simulink model "ASM_Traffic_MultiCore"  (R2026a)
settings: Solver=ode1  StartTime=SIM.tstart.v  StopTime=SIM.tend.v  FixedStep=SIM.StepSize.v
PostLoadFcn:
  | if any(exist('dsrtsu_mdlpostloadfcn', 'file') ~= 0), dsrtsu_mdlpostloadfcn('Execute', bdroot); end
  | try, asm_mdl_postloadfcn(bdroot, 'UpdateModel', 3600); catch, disp(lasterr); end,
InitFcn:
  | , if any(exist('rtifpga_mdlclblib', 'file') ~= 0), rtifpga_mdlclblib('Init', bdroot); end,
  | , if any(exist('dsmpb_private', 'file') ~= 0), dsmpb_private('dsmpb_mdlclblib', 'Init', bdroot); end,
model workspace (MAT data in the model file):
  asmReferencePath = [0 0.01 0.02 0.03 0.04 0.05 0.06 0.07 0.08 0.09 0.1 0.11 ... (350007 elements, 50001x7)]
  roadBounds : Simulink.Parameter (value not decoded)
  safetyAxes : Simulink.Parameter (value not decoded)
undefined symbols (not defined in the file): _to_, a0b2, ASM_BrakeHydraulics_DemoSystems, ASM_VehicleDynamics_DemoSystems, b98103fe8ad365046cd0, BrakeCircuit, controllerConfig, CPT, Crankshaft, DiscIntNeverNeededParam, dsmsi, FinalDriveAssembly, MDL, ModeSignals, mu, Pos_BrakePedal_Maneuver, rad, RefSignals, roadFamilyData, roadFamilyId, s_to_rpm, SIM, SoftECU, Suspension, Tire, Transmission
libraries: ASM_Traffic_lib x135, simulink x98, ASM_Utils_lib x77, ASM_VehicleDynamics_lib x70, ASM_Environment_lib x22, dsmpblib x20, dsmsilib x15, MDLD_Utils_lib x10, ASM_BrakeHydraulics_lib x3, sl_discontinuities x2
(part 35 of 65)

== system ASM_Traffic_MultiCore/VehicleDynamics/SignalInterface/ExternalOutports/Select_Outport_Signals ==
  ASMSignalBus : Inport
  Bus Selector : BusSelector  OutputSignals=VehicleMovement.Accelerations.VehicleCoG.Linear.a_Vehicle_CoG[x;y;z][m|s2].a_x_Vehicle_CoG[m|s2],VehicleMovement.Accelerations.VehicleCoG.Linear.a_Vehicle_CoG[x;y;z][m|s2].a_y_Vehicle_CoG[m|s2],VehicleMovement.Accelerations.VehicleCoG.Linear.a_Vehicle_CoG[x;y;z][m|s2].a_z_Vehicle_CoG[m|s2],VehicleMovement.Velocities.Vehicle.Linear.v_Vehicle_CoG[x;y;z][km|h].v_x_Vehicle_CoG[km|h],VehicleMovement.Velocities.Vehicle.Linear.v_Vehicle_CoG[x;y;z][km|h].v_y_Vehicle_CoG[km|h],VehicleMovement.Velocities.Vehicle.Linear.v_Vehicle_CoG[x;y;z][km|h].v_z_Vehicle_CoG[km|h],VehicleMovement.Velocities.Vehicle.Linear.v_Total_Vehicle[km|h],VehicleMovement.Velocities.Vehicle.Linear.Angle_SideSlip_Vehicle[deg],VehicleMovement.Velocities.Vehicle.Angular.w_Vehicle_CoG[x;y;z][deg|s].RollRate_Vehicle_CoG[deg|s],VehicleMovement.Velocities.Vehicle.Angular.w_Vehicle_CoG[x;y;z][deg|s].PitchRate_Vehicle_CoG[deg|s],VehicleMovement.Velocities.Vehicle.Angular.w_Vehicle_CoG[x;y;z][deg|s].YawRate_Vehicle_CoG[deg|s],VehicleMovement.Positions.Vehicle.Linear.Pos_Vehicle_CoorSys_E[x;y;z][m].Pos_x_Vehicle_CoorSys_E[m],VehicleMovement.Positions.Vehicle.Linear.Pos_Vehicle_CoorSys_E[x;y;z][m].Pos_y_Vehicle_CoorSys_E[m],VehicleMovement.Positions.Vehicle.Linear.Pos_Vehicle_CoorSys_E[x;y;z][m].Pos_z_Vehicle_CoorSys_E[m],VehicleMovement.Positions.Vehicle.Linear.Pos_Vehicle_CoorSys_E[m],VehicleMovement.Positions.Vehicle.Linear.s_Vehicle[m],VehicleMovement.Positions.Vehicle.Angular.Angle_Vehicle_CoorSys_E[x;y;z][deg].Angle_Roll_Vehicle_CoorSys_E[deg],VehicleMovement.Positions.Vehicle.Angular.Angle_Vehicle_CoorSys_E[x;y;z][deg].Angle_Pitch_Vehicle_CoorSys_E[deg],VehicleMovement.Positions.Vehicle.Angular.Angle_Vehicle_CoorSys_E[x;y;z][deg].Angle_Yaw_Vehicle_CoorSys_E[deg],VehicleMovement.VehicleMassAndAdditionalLoads.m_TotalVehicle[kg],VehicleMovement.VehicleMassAndAdditionalLoads.PosVec_CoG_TotalVehicle[x;y;z][m]  OutputAsBus=on
  Bus Selector1 : BusSelector  OutputSignals=Wheel.WheelSpeed  OutputAsBus=on
  Bus Selector2 : BusSelector  OutputSignals=Brake.BrakeDisc.Pressure,Brake.BrakeDisc.Const_BrakeDiscFactor,Brake.BrakeDisc.Torque  OutputAsBus=on
  Bus Selector3 : BusSelector  OutputSignals=Steering.StatesSteeringSystem,Steering.SteeringWheelTorque,Steering.ForcesAndTorques,Steering.i_Steering_Mean[]  OutputAsBus=on
  Bus Selector4 : BusSelector  OutputSignals=Tire.r_Dyn_Tire[FL;FR;RL;RR][m],Tire.r_Dyn_Tire_Mean[m],Tire.Coef_RollingRes[FL;FR;RL;RR][],Tire.Coef_RollingRes_Mean[],Tire.CorneringStiffness_Tire_Front[N|rad],Tire.CorneringStiffness_Tire_Rear[N|rad],Tire.CorneringStiffness[FL;FR;RL;RR][N|rad]  OutputAsBus=on
  Bus Selector5 : BusSelector  OutputSignals=Suspension.SuspensionFront.RelativePositionFront.Pos_Wheel[FL;FR][x;y;z][m],Suspension.SuspensionRear.RelativePositionRear.Pos_Wheel[RL;RR][x;y;z][m],Suspension.SuspensionFront.SuspensionKinematicsFront,Suspension.SuspensionRear.SuspensionKinematicsRear  OutputAsBus=on
  Bus Selector6 : BusSelector  OutputSignals=Aerodynamics  OutputAsBus=on
  Vehicle_Movement : Outport  VectorParamsAs1DForOutWhenUnconnected=off
  Tire : Outport  Port=2  VectorParamsAs1DForOutWhenUnconnected=off
  WheelSpeed : Outport  Port=3  VectorParamsAs1DForOutWhenUnconnected=off
  Brake : Outport  Port=4  VectorParamsAs1DForOutWhenUnconnected=off
  Steering : Outport  Port=5  VectorParamsAs1DForOutWhenUnconnected=off
  Suspension : Outport  Port=6  VectorParamsAs1DForOutWhenUnconnected=off
  Aerodynamics : Outport  Port=7  VectorParamsAs1DForOutWhenUnconnected=off
  wires:
  Bus Selector3/1 -> Steering/1
  Bus Selector2/1 -> Brake/1
  Bus Selector1/1 -> WheelSpeed/1
  Bus Selector/1 -> Vehicle_Movement/1
  Bus Selector4/1 -> Tire/1
  ASMSignalBus/1 -> Bus Selector/1, Bus Selector4/1, Bus Selector1/1, Bus Selector6/1, Bus Selector5/1, Bus Selector3/1, Bus Selector2/1
  Bus Selector6/1 -> Aerodynamics/1
  Bus Selector5/1 -> Suspension/1

== system ASM_Traffic_MultiCore/AnimationInterface/ANIMATION_INTERFACE/Connection_Settings/Ethernet_TCP/HIL ==
  Tx_Length : Inport
  Tx_Data : Inport  Port=2
  Receive [ETH TCP (Server)\Connection 1] : dsmpblib/Data Inport  Priority=10000
      settings: SourceProductName=dSPACE Model Interface Package for Simulink (MIPS)
  Status [ETH TCP (Server)\Connection 1] : dsmpblib/Data Inport  Priority=10000
      settings: SourceProductName=dSPACE Model Interface Package for Simulink (MIPS)
  Transmit_In [ETH TCP (Server)\Connection 1] : dsmpblib/Data Inport  Priority=10000
      settings: SourceProductName=dSPACE Model Interface Package for Simulink (MIPS)
  Transmit_Out [ETH TCP (Server)\Connection 1] : dsmpblib/Data Outport  Priority=20000
      settings: SourceProductName=dSPACE Model Interface Package for Simulink (MIPS)
  Connected : Outport
  Tx_Sent_bytes : Outport  Port=2
  Rx_Length : Outport  Port=3
  Rx_Data : Outport  Port=4
  wires:
  Tx_Length/1 -> Transmit_Out [ETH TCP (Server)\Connection 1]/1
  Tx_Data/1 -> Transmit_Out [ETH TCP (Server)\Connection 1]/2
  Status [ETH TCP (Server)\Connection 1]/1 -> Connected/1
  Transmit_In [ETH TCP (Server)\Connection 1]/1 -> Tx_Sent_bytes/1
  Receive [ETH TCP (Server)\Connection 1]/1 -> Rx_Length/1
  Receive [ETH TCP (Server)\Connection 1]/2 -> Rx_Data/1

== system ASM_Traffic_MultiCore/AnimationInterface/ANIMATION_INTERFACE/Connection_Settings/Ethernet_TCP/SIL ==
  Tx_Length : Inport
  Tx_Data : Inport  Port=2
  Connected_ : Constant  OutDataTypeStr=Inherit: Inherit via back propagation
  Data Type Conversion : DataTypeConversion  OutDataTypeStr=uint32  SaturateOnIntegerOverflow=off  RndMeth=Floor
  Display : Display
      settings: Format=decimal (Stored Integer)
  dsmsi_eth_tcp_server_BL1 : dsmsilib/Utilities/dsmsi_eth_tcp_server_BL1  paramPort=2017  paramMaximumRxMessageSize=65507  paramBlocking=0  paramEnableReconnectPort=off  paramEnableMaxRxLength=off
      settings: SourceProductName=dSPACE MSI Blockset
  Connected : Outport
  Tx_Sent_bytes : Outport  Port=2
  Rx_Length : Outport  Port=3
  Rx_Data : Outport  Port=4
  wires:
  Data Type Conversion/1 -> Rx_Length/1
  dsmsi_eth_tcp_server_BL1/3 -> Data Type Conversion/1
  Connected_/1 -> Connected/1
  dsmsi_eth_tcp_server_BL1/2 -> Tx_Sent_bytes/1
  dsmsi_eth_tcp_server_BL1/4 -> Rx_Data/1
  dsmsi_eth_tcp_server_BL1/1 -> Display/1
  Tx_Length/1 -> dsmsi_eth_tcp_server_BL1/1
  Tx_Data/1 -> dsmsi_eth_tcp_server_BL1/2

== system ASM_Traffic_MultiCore/AnimationInterface/ANIMATION_INTERFACE/Sensors/Object_Sensor_2D_Points/Calc_Object_Sensor_2D_Points ==
  Transform_In : Inport
  ModelSignals : Inport  Port=2
  Bus Selector2 : BusSelector  OutputSignals=Angle_Hor_Rel[deg],Distance[m],Num_SensorRays_Used[]
  Sensor_Points : Subsystem
  AnimationSignals : Outport  VectorParamsAs1DForOutWhenUnconnected=off
  wires:
  ModelSignals/1 -> Bus Selector2/1
  Transform_In/1 -> Sensor_Points/1(Transform_In)
  Bus Selector2/2 -> Sensor_Points/3(Distance[m])  "<Distance[m]>"
  Sensor_Points/1(Translate[x;y;z][m]) -> AnimationSignals/1
  Bus Selector2/3 -> Sensor_Points/4(Num_SensorRays_Used[])  "<Num_SensorRays_Used[]>"
  Bus Selector2/1 -> Sensor_Points/2(Angle_Hor_Rel[deg])  "<Angle_Hor_Rel[deg]>"

== system ASM_Traffic_MultiCore/AnimationInterface/ANIMATION_INTERFACE/Sensors/Object_Sensor_2D_Points/Object_Sensor_2D_Transformation1 ==
  Transform_In1 : Inport
  ModelSignals : Inport  Port=2
  Bus Selector1 : BusSelector  OutputSignals=Pos_Sensor_Apex_CoorSys_V[x;y;z][m],Angle_z_Orientation_Sensor_CoorSys_V[deg]
  Mux : Mux  Inputs=3
  SensorApex : dsmsilib/dsmsi_simulation_data_objects_BL1  Priority=10001  parameterStr="{\"Version\":1,\"TransformInput\":false,\"EnableInput\":false,\"Objects\":[{\"Name\":\"SensorApex\",\"TypeClass\":{\"Name\":\"Transformation\",\"Class\":1,\"SignalProperty\":null,\"TransformationProperty\":{\"TransformMatrixIn\":true,\"TransformMatrixOut\":true,\"AngleInterpretation\":0,\"TransformationOrder\":0,\"RotationOrder\":0,\"TranslationAsParameter\":false,\"Translation\":\"[0 0 0]\",\"RotationAsParameter\":false,\"Rotation\":\"[0 0 0]\",\"ScalingAsParameter\":true,\"Scaling\":\"[1 1 1]\",\"ObjectsCount\":1},\"PositionAndScaleProperty\":null,\"PositionProperty\":null},\"Children\":[],\"Oid\":1}]}"  evalStr=dsmsi(gcb, 'EvalJson')  sampleTime=-1  globalBlockId=0  objectsBlockId=dsmsi(gcb, 'GetObjectBlockId')  objectsBlockGuiOpen=dsmsi(gcb, 'GetSdoGuiStatus')  dialogIsOpen=0  blockVersion=60  highPrecision=0  validNameBckp=SensorApex
      settings: SourceProductName=dSPACE MSI Blockset
  zero : Constant  Value=0
  Transform_Out : Outport  VectorParamsAs1DForOutWhenUnconnected=off
  wires:
  SensorApex/1 -> Transform_Out/1
  Mux/1 -> SensorApex/3
  Bus Selector1/1 -> SensorApex/2  "<Pos_Sensor_Apex_CoorSys_V[x;y;z][m]>"
  Transform_In1/1 -> SensorApex/1
  ModelSignals/1 -> Bus Selector1/1
  zero/1 -> Mux/3, Mux/2
  Bus Selector1/2 -> Mux/1  "<Angle_z_Orientation_Sensor_CoorSys_V[deg]>"

== system ASM_Traffic_MultiCore/AnimationInterface/ANIMATION_INTERFACE/Sensors/Object_Sensor_3D_CustomPoints/AdaptPointSensor1_To_Dim_60 ==
  ID[] : Inport
  Pos_ObjectPoint_CoorSys_E[x;y;z][m] : Inport  Port=2
  Demux1 : Demux  Outputs=3
  Mux1 : Mux  Inputs=3
  Select_1_60_{1..4} (4 alike) : Selector  InputPortWidth=MDL.Traffic.Sensors.CustomPoints_1.Const_Output_Dimension_Object_Points.v*MDL.Traffic.Sensors.CustomPoints_1.Const_Output_Dimension_Objects.v  IndexOptions=Index vector (dialog)  Indices=[1:60]  OutputSizes=1
  ID_Adatpted[] : Outport  VectorParamsAs1DForOutWhenUnconnected=off
  Pos_ObjectPoint_CoorSys_E_Adapted[x;y;z][m] : Outport  Port=2  VectorParamsAs1DForOutWhenUnconnected=off
  wires:
  Mux1/1 -> Pos_ObjectPoint_CoorSys_E_Adapted[x;y;z][m]/1
  Demux1/3 -> Select_1_60_4/1
  Select_1_60_4/1 -> Mux1/3
  Select_1_60_3/1 -> Mux1/2
  Demux1/2 -> Select_1_60_3/1
  Demux1/1 -> Select_1_60_2/1
  Select_1_60_2/1 -> Mux1/1
  Select_1_60_1/1 -> ID_Adatpted[]/1
  ID[]/1 -> Select_1_60_1/1
  Pos_ObjectPoint_CoorSys_E[x;y;z][m]/1 -> Demux1/1

== system ASM_Traffic_MultiCore/AnimationInterface/ANIMATION_INTERFACE/Sensors/Object_Sensor_3D_CustomPoints/AdaptPointSensor2_To_Dim_60 ==
  ID[] : Inport
  Pos_ObjectPoint_CoorSys_E[x;y;z][m] : Inport  Port=2
  Demux1 : Demux  Outputs=3
  Mux1 : Mux  Inputs=3
  Select_1_60_{1..4} (4 alike) : Selector  InputPortWidth=MDL.Traffic.Sensors.CustomPoints_2.Const_Output_Dimension_Object_Points.v*MDL.Traffic.Sensors.CustomPoints_2.Const_Output_Dimension_Objects.v  IndexOptions=Index vector (dialog)  Indices=[1:60]  OutputSizes=1
  ID_Adatpted[] : Outport  VectorParamsAs1DForOutWhenUnconnected=off
  Pos_ObjectPoint_CoorSys_E_Adapted[x;y;z][m] : Outport  Port=2  VectorParamsAs1DForOutWhenUnconnected=off
  wires:
  Select_1_60_4/1 -> Mux1/3
  Select_1_60_3/1 -> Mux1/2
  Select_1_60_2/1 -> Mux1/1
  Select_1_60_1/1 -> ID_Adatpted[]/1
  Demux1/1 -> Select_1_60_2/1
  Mux1/1 -> Pos_ObjectPoint_CoorSys_E_Adapted[x;y;z][m]/1
  Pos_ObjectPoint_CoorSys_E[x;y;z][m]/1 -> Demux1/1
  ID[]/1 -> Select_1_60_1/1
  Demux1/3 -> Select_1_60_4/1
  Demux1/2 -> Select_1_60_3/1

== system ASM_Traffic_MultiCore/AnimationInterface/ANIMATION_INTERFACE/Sensors/Object_Sensor_3D_CustomPoints/AdaptPointSensor3_To_Dim_60 ==
  ID[] : Inport
  Pos_ObjectPoint_CoorSys_E[x;y;z][m] : Inport  Port=2
  Demux1 : Demux  Outputs=3
  Mux1 : Mux  Inputs=3
  Select_1_60_{1..4} (4 alike) : Selector  InputPortWidth=MDL.Traffic.Sensors.CustomPoints_3.Const_Output_Dimension_Object_Points.v*MDL.Traffic.Sensors.CustomPoints_3.Const_Output_Dimension_Objects.v  IndexOptions=Index vector (dialog)  Indices=[1:60]  OutputSizes=1
  ID_Adatpted[] : Outport  VectorParamsAs1DForOutWhenUnconnected=off
  Pos_ObjectPoint_CoorSys_E_Adapted[x;y;z][m] : Outport  Port=2  VectorParamsAs1DForOutWhenUnconnected=off
  wires:
  Select_1_60_4/1 -> Mux1/3
  Select_1_60_3/1 -> Mux1/2
  Select_1_60_2/1 -> Mux1/1
  Select_1_60_1/1 -> ID_Adatpted[]/1
  Demux1/2 -> Select_1_60_3/1
  Demux1/3 -> Select_1_60_4/1
  ID[]/1 -> Select_1_60_1/1
  Pos_ObjectPoint_CoorSys_E[x;y;z][m]/1 -> Demux1/1
  Mux1/1 -> Pos_ObjectPoint_CoorSys_E_Adapted[x;y;z][m]/1
  Demux1/1 -> Select_1_60_2/1

== system ASM_Traffic_MultiCore/AnimationInterface/ANIMATION_INTERFACE/Sensors/Object_Sensor_3D_RadarEffect_Points/AdaptPointDimensionSensor1 ==
  ID[] : Inport
  Pos_ObjectPoint_CoorSys_E[x;y;z][m] : Inport  Port=2
  Demux1 : Demux  Outputs=3
  Mux1 : Mux  Inputs=3
  Selector{1..4} (4 alike) : Selector  InputPortWidth=MDL.Traffic.Sensors.RadarReflectionPoints_1.Const_Output_Dimension_Objects.v*MDL.Traffic.Sensors.RadarReflectionPoints_1.Const_Output_Dimension_Object_Points.v  IndexOptions=Index vector (dialog)  Indices=[1:60]  OutputSizes=1
  ID_Adatpted[] : Outport  VectorParamsAs1DForOutWhenUnconnected=off
  Pos_ObjectPoint_CoorSys_E_Adapted[x;y;z][m] : Outport  Port=2  VectorParamsAs1DForOutWhenUnconnected=off
  wires:
  Pos_ObjectPoint_CoorSys_E[x;y;z][m]/1 -> Demux1/1
  ID[]/1 -> Selector3/1
  Selector3/1 -> ID_Adatpted[]/1
  Selector1/1 -> Mux1/1
  Demux1/1 -> Selector1/1
  Demux1/2 -> Selector2/1
  Selector2/1 -> Mux1/2
  Selector4/1 -> Mux1/3
  Demux1/3 -> Selector4/1
  Mux1/1 -> Pos_ObjectPoint_CoorSys_E_Adapted[x;y;z][m]/1

== system ASM_Traffic_MultiCore/AnimationInterface/ANIMATION_INTERFACE/Sensors/Object_Sensor_3D_RadarEffect_Points/AdaptPointDimensionSensor2 ==
  ID[] : Inport
  Pos_ObjectPoint_CoorSys_E[x;y;z][m] : Inport  Port=2
  Demux1 : Demux  Outputs=3
  Mux1 : Mux  Inputs=3
  Selector{1..4} (4 alike) : Selector  InputPortWidth=MDL.Traffic.Sensors.RadarReflectionPoints_2.Const_Output_Dimension_Objects.v*MDL.Traffic.Sensors.RadarReflectionPoints_2.Const_Output_Dimension_Object_Points.v  IndexOptions=Index vector (dialog)  Indices=[1:60]  OutputSizes=1
  ID_Adatpted[] : Outport  VectorParamsAs1DForOutWhenUnconnected=off
  Pos_ObjectPoint_CoorSys_E_Adapted[x;y;z][m] : Outport  Port=2  VectorParamsAs1DForOutWhenUnconnected=off
  wires:
  Mux1/1 -> Pos_ObjectPoint_CoorSys_E_Adapted[x;y;z][m]/1
  Demux1/3 -> Selector4/1
  Selector4/1 -> Mux1/3
  Selector2/1 -> Mux1/2
  Demux1/2 -> Selector2/1
  Demux1/1 -> Selector1/1
  Selector1/1 -> Mux1/1
  Selector3/1 -> ID_Adatpted[]/1
  ID[]/1 -> Selector3/1
  Pos_ObjectPoint_CoorSys_E[x;y;z][m]/1 -> Demux1/1

== system ASM_Traffic_MultiCore/AnimationInterface/ANIMATION_INTERFACE/Sensors/Object_Sensor_3D_RadarEffect_Points/AdaptPointDimensionSensor3 ==
  ID[] : Inport
  Pos_ObjectPoint_CoorSys_E[x;y;z][m] : Inport  Port=2
  Demux1 : Demux  Outputs=3
  Mux1 : Mux  Inputs=3
  Selector{1..4} (4 alike) : Selector  InputPortWidth=MDL.Traffic.Sensors.RadarReflectionPoints_3.Const_Output_Dimension_Objects.v*MDL.Traffic.Sensors.RadarReflectionPoints_3.Const_Output_Dimension_Object_Points.v  IndexOptions=Index vector (dialog)  Indices=[1:60]  OutputSizes=1
  ID_Adatpted[] : Outport  VectorParamsAs1DForOutWhenUnconnected=off
  Pos_ObjectPoint_CoorSys_E_Adapted[x;y;z][m] : Outport  Port=2  VectorParamsAs1DForOutWhenUnconnected=off
  wires:
  Pos_ObjectPoint_CoorSys_E[x;y;z][m]/1 -> Demux1/1
  ID[]/1 -> Selector3/1
  Selector3/1 -> ID_Adatpted[]/1
  Selector1/1 -> Mux1/1
  Demux1/1 -> Selector1/1
  Demux1/2 -> Selector2/1
  Selector2/1 -> Mux1/2
  Selector4/1 -> Mux1/3
  Demux1/3 -> Selector4/1
  Mux1/1 -> Pos_ObjectPoint_CoorSys_E_Adapted[x;y;z][m]/1

== system ASM_Traffic_MultiCore/DomainControl/DriverAssistance/Control/SoftECU_ACC/Soft_ECU_ACC ==
  Switches_ACC_User : Inport
  v_x_Vehicle_CoG[km|h] : Inport  Port=2
  YawRate_Vehicle_CoG[deg|s] : Inport  Port=3
  Pos_FL_Wheel[x;y;z][m] : Inport  Port=4
  Pos_FR_Wheel[x;y;z][m] : Inport  Port=5
  r_Dyn_Tire[FL;FR;RL;RR][m] : Inport  Port=6
  Coef_RollingRes[FL;FR;RL;RR][] : Inport  Port=7
  Cw_x[] : Inport  Port=8
  i_FrontDrive[] : Inport  Port=9
  i_RearDrive[] : Inport  Port=10
  TrqDistri_Front_Rear[0_1] : Inport  Port=11
  i_unsync_Trm[] : Inport  Port=12
  m_TotalVehicle[kg] : Inport  Port=13
  Trq_Fric_Engine[Nm] : Inport  Port=14
  Pos_AccPedal[%] : Inport  Port=15
  Pos_BrakePedal[%] : Inport  Port=16
  Slope_Veh_Road[%] : Inport  Port=17
  s_Vehicle_Road[m] : Inport  Port=18
  d_Vehicle_Road[m] : Inport  Port=19
  Dist_Fellows[m] : Inport  Port=20
  v_Rel_Fellows[m|s] : Inport  Port=21
  Angle_Hor_Rel_Fellows[deg] : Inport  Port=22
  s_Fellows_Ref[m] : Inport  Port=23
  d_Total_Fellows[m] : Inport  Port=24
  PosVec_MainPnt_Fellows[x;y;z][m] : Inport  Port=25
  Length_Fellows[m] : Inport  Port=26
  Width_Fellows[m] : Inport  Port=27
  Height_Fellows[m] : Inport  Port=28
  Object_ID[] : Inport  Port=29
  ECU_Commands[] : Inport  Port=30
  Reset[0|1] : Inport  Port=31
  ASMSignalCollector : Subsystem
  CONTROLLER_ACC : ASM_Traffic_lib/SoftECU/CONTROLLER_ACC  Tag=ASM_SUBCOMPONENT  Const_Kp_Dist_Ctrl=MDL.SoftECU.ACC.Const_Kp_Dist_Ctrl  Const_Ki_Dist_Ctrl=MDL.SoftECU.ACC.Const_Ki_Dist_Ctrl  Const_Kp_v_Ctrl=MDL.SoftECU.ACC.Const_Kp_v_Ctrl  Const_Ki_v_Ctrl=MDL.SoftECU.ACC.Const_Ki_v_Ctrl  Map_a_UpperLimit=MDL.SoftECU.ACC.Map_a_UpperLimit  Map_a_LowerLimit=MDL.SoftECU.ACC.Map_a_LowerLimit  Const_v_Threshold=MDL.SoftECU.ACC.Const_v_Threshold  Const_Dist_Threshold=MDL.SoftECU.ACC.Const_Dist_Threshold  Map_a_RisingRateMax=MDL.SoftECU.ACC.Map_a_RisingRateMax  Map_a_FallingRateMax=MDL.SoftECU.ACC.Map_a_FallingRateMax  Const_a_Max_AEB=MDL.SoftECU.ACC.Const_a_Max_AEB  Const_Response_Time_FCW=MDL.SoftECU.ACC.Const_Response_Time_FCW  Const_Dist_Min_Set=MDL.SoftECU.ACC.Const_Dist_Min_Set  Map_TTCThresholdAEB=MDL.SoftECU.ACC.Map_TTCThresholdAEB  StepSize=SIM.StepSize  ASMProperties=struct('Name','CONTROLLER_ACC','Version','9.0','Library','ASM_Traffic_lib')  ASMInstanceName=controller_acc  ASMInstanceID=1
  ControlModel_Signals : Subsystem
  Goto Tag Visibility : GotoTagVisibility  GotoTag=ASMBUS_SoftECU_ACC_Target_Selection
  Goto Tag Visibility1 : GotoTagVisibility  GotoTag=ASMBUS_SoftECU_ACC_Controller
  Goto Tag Visibility2 : GotoTagVisibility  GotoTag=ASMBUS_SoftECU_ACC_User_Interface
  Goto Tag Visibility3 : GotoTagVisibility  GotoTag=ASMBUS_SoftECU_ACC_Interface
  Input_Selection : Subsystem
  Map_Inputs : Subsystem
  Mux : Mux  Inputs=2
  OUTPUT_INTERFACE_ACC : ASM_Traffic_lib/SoftECU/OUTPUT_INTERFACE_ACC  Tag=ASM_SUBCOMPONENT  ASMProperties=struct('Name','OUTPUT_INTERFACE_ACC','Version','5.0','Library','ASM_Traffic_lib')  ASMInstanceName=output_interface_acc  ASMInstanceID=1
  Rate Transition : RateTransition  Integrity=off  OutPortSampleTimeOpt=Inherit
  Rate Transition1 : RateTransition  Integrity=off  OutPortSampleTimeOpt=Inherit
  Sw_ACC_Distance[s] : Constant  Value=2
  TARGET_SELECTION_ACC : ASM_Traffic_lib/SoftECU/TARGET_SELECTION_ACC  Tag=ASM_SUBCOMPONENT  Const_Dist_SafetyBound=MDL.SoftECU.ACC.Const_Dist_SafetyBound  Sw_LaneCrossingCheck=MDL.SoftECU.ACC.Sw_LaneCrossingCheck  StepSize=SIM.StepSize  ASMProperties=struct('Name','TARGET_SELECTION_ACC','Version','6.0','Library','ASM_Traffic_lib')  ASMInstanceName=target_selection_acc  ASMInstanceID=1
  Tire : Subsystem
  TrackWidthVehicle : Subsystem
  USER_INTERFACE_ACC : ASM_Traffic_lib/SoftECU/USER_INTERFACE_ACC  Tag=ASM_SUBCOMPONENT  Const_v_Step=MDL.SoftECU.ACC.Const_v_Step_CC  ASMProperties=struct('Name','USER_INTERFACE_ACC','Version','6.0','Library','ASM_Traffic_lib')  ASMInstanceName=user_interface_acc  ASMInstanceID=1
  avoid_incomplete_trace2source : Subsystem
  avoid_incomplete_trace2source1 : Subsystem
  avoid_incomplete_trace2source10 : Subsystem
  avoid_incomplete_trace2source2 : Subsystem
  avoid_incomplete_trace2source4 : Subsystem
  avoid_incomplete_trace2source5 : Subsystem
  avoid_incomplete_trace2source6 : Subsystem
  avoid_incomplete_trace2source7 : Subsystem
  avoid_incomplete_trace2source8 : Subsystem
  avoid_incomplete_trace2source9 : Subsystem
  hide_algebraic_loop : UnitDelay  SampleTime=-1
  hide_algebraic_loop1 : UnitDelay  SampleTime=-1
  "hide_algebraic_loop2 " : UnitDelay  SampleTime=-1
  ASMSignalBus : Outport  VectorParamsAs1DForOutWhenUnconnected=off
  Enable_Trq_Engine_ACC[0|1] : Outport  Port=2  VectorParamsAs1DForOutWhenUnconnected=off
  Trq_Request_Engine_ACC[Nm] : Outport  Port=3  VectorParamsAs1DForOutWhenUnconnected=off
  Trq_Request_Engine_ACC[Front;Rear][Nm] : Outport  Port=4  VectorParamsAs1DForOutWhenUnconnected=off
  Enable_Trq_Brake_ACC[0|1] : Outport  Port=5  VectorParamsAs1DForOutWhenUnconnected=off
  Trq_Request_Brake_ACC[Nm] : Outport  Port=6  VectorParamsAs1DForOutWhenUnconnected=off
  FCW[0|1] : Outport  Port=7  VectorParamsAs1DForOutWhenUnconnected=off
  AEB[0|1] : Outport  Port=8  VectorParamsAs1DForOutWhenUnconnected=off
  ACC_State[1OFF|2Standby|3ON] : Outport  Port=9  VectorParamsAs1DForOutWhenUnconnected=off
  Driver_Override_ACC_Active[0Off|1On] : Outport  Port=10  VectorParamsAs1DForOutWhenUnconnected=off
  Driver_Override_ACC_Reason[0NoOverride|1BrakePedal|2AccPedal] : Outport  Port=11  VectorParamsAs1DForOutWhenUnconnected=off
  tag scope: ASMBUS_SoftECU_ACC_Controller=scoped, ASMBUS_SoftECU_ACC_Interface=scoped, ASMBUS_SoftECU_ACC_Target_Selection=scoped, ASMBUS_SoftECU_ACC_User_Interface=scoped
  wires:
  avoid_incomplete_trace2source10/1(Out1) -> USER_INTERFACE_ACC/10
  Map_Inputs/7(Sw_ACC_Speed_Decrease[0Off|1On]) -> avoid_incomplete_trace2source10/1(In1)
  avoid_incomplete_trace2source9/1(Out1) -> USER_INTERFACE_ACC/9
  Map_Inputs/6(Sw_ACC_Speed_Increase[0Off|1On]) -> avoid_incomplete_trace2source9/1(In1)
  avoid_incomplete_trace2source8/1(Out1) -> USER_INTERFACE_ACC/8
  Map_Inputs/5(Sw_ACC_Speed_Set[0Off|1On]) -> avoid_incomplete_trace2source8/1(In1)
  avoid_incomplete_trace2source7/1(Out1) -> USER_INTERFACE_ACC/7
  Map_Inputs/4(Sw_ACC_Resume[0Off|1On]) -> avoid_incomplete_trace2source7/1(In1)
  avoid_incomplete_trace2source6/1(Out1) -> USER_INTERFACE_ACC/6
  Map_Inputs/3(Sw_ACC_Cancel[0Off|1On]) -> avoid_incomplete_trace2source6/1(In1)
  avoid_incomplete_trace2source5/1(Out1) -> USER_INTERFACE_ACC/5
  Map_Inputs/2(Sw_ACC_Off[0Off|1On]) -> avoid_incomplete_trace2source5/1(In1)
  avoid_incomplete_trace2source4/1(Out1) -> USER_INTERFACE_ACC/4
  Map_Inputs/1(Sw_ACC_On[0Off|1On]) -> avoid_incomplete_trace2source4/1(In1)
  Sw_ACC_Distance[s]/1 -> CONTROLLER_ACC/10
  avoid_incomplete_trace2source2/1(Out1) -> CONTROLLER_ACC/9
  Map_Inputs/8(Sw_ACC_BrakeMode[1Comfort|2AEBOnly|3AEBOff]) -> avoid_incomplete_trace2source2/1(In1)
  avoid_incomplete_trace2source1/1(Out1) -> CONTROLLER_ACC/8
  USER_INTERFACE_ACC/3 -> avoid_incomplete_trace2source1/1(In1)
  avoid_incomplete_trace2source/1(Out1) -> CONTROLLER_ACC/7
  USER_INTERFACE_ACC/2 -> avoid_incomplete_trace2source/1(In1)
  CONTROLLER_ACC/6 -> AEB[0|1]/1
  CONTROLLER_ACC/5 -> FCW[0|1]/1
  Trq_Fric_Engine[Nm]/1 -> OUTPUT_INTERFACE_ACC/10
  Coef_RollingRes[FL;FR;RL;RR][]/1 -> Tire/2(Coef_RollingRes[FL;FR;RL;RR][])
  r_Dyn_Tire[FL;FR;RL;RR][m]/1 -> Tire/1(r_Dyn_Tire[FL;FR;RL;RR][m])
  CONTROLLER_ACC/1 -> [ASMBUS_SoftECU_ACC_Controller]
  ASMSignalCollector/1(ASMSignalBus) -> ASMSignalBus/1
  Tire/1(r_Dyn_Tire_Mean[m]) -> OUTPUT_INTERFACE_ACC/2
  Tire/2(Coef_RollingRes_Mean[]) -> OUTPUT_INTERFACE_ACC/3
  Cw_x[]/1 -> OUTPUT_INTERFACE_ACC/4
  Slope_Veh_Road[%]/1 -> OUTPUT_INTERFACE_ACC/8
  v_x_Vehicle_CoG[km|h]/1 -> TARGET_SELECTION_ACC/2, USER_INTERFACE_ACC/1, CONTROLLER_ACC/1, OUTPUT_INTERFACE_ACC/9
  OUTPUT_INTERFACE_ACC/3 -> Trq_Request_Engine_ACC[Nm]/1
  OUTPUT_INTERFACE_ACC/2 -> Trq_Request_Brake_ACC[Nm]/1
  OUTPUT_INTERFACE_ACC/1 -> [ASMBUS_SoftECU_ACC_Interface]
  i_unsync_Trm[]/1 -> OUTPUT_INTERFACE_ACC/6
  m_TotalVehicle[kg]/1 -> OUTPUT_INTERFACE_ACC/7
  YawRate_Vehicle_CoG[deg|s]/1 -> TARGET_SELECTION_ACC/1
  CONTROLLER_ACC/2 -> hide_algebraic_loop/1
  TARGET_SELECTION_ACC/1 -> [ASMBUS_SoftECU_ACC_Target_Selection]
  Mux/1 -> OUTPUT_INTERFACE_ACC/5
  USER_INTERFACE_ACC/1 -> [ASMBUS_SoftECU_ACC_User_Interface]
  Switches_ACC_User/1 -> Map_Inputs/2(Switches_ACC_User)
  ECU_Commands[]/1 -> Map_Inputs/3(ECU_Commands[])
  TARGET_SELECTION_ACC/4 -> CONTROLLER_ACC/4
  TARGET_SELECTION_ACC/3 -> CONTROLLER_ACC/3
  TARGET_SELECTION_ACC/2 -> Rate Transition/1
  Rate Transition/1 -> CONTROLLER_ACC/2
  CONTROLLER_ACC/3 -> hide_algebraic_loop1/1
  CONTROLLER_ACC/4 -> "hide_algebraic_loop2 "/1
  hide_algebraic_loop1/1 -> Enable_Trq_Engine_ACC[0|1]/1, OUTPUT_INTERFACE_ACC/11
  "hide_algebraic_loop2 "/1 -> Enable_Trq_Brake_ACC[0|1]/1, OUTPUT_INTERFACE_ACC/12
  hide_algebraic_loop/1 -> OUTPUT_INTERFACE_ACC/1
  Pos_AccPedal[%]/1 -> USER_INTERFACE_ACC/2
  Pos_BrakePedal[%]/1 -> USER_INTERFACE_ACC/3
  Pos_FL_Wheel[x;y;z][m]/1 -> TrackWidthVehicle/1(Pos_FL_Wheel[x;y;z][m])
  Pos_FR_Wheel[x;y;z][m]/1 -> TrackWidthVehicle/2(Pos_FR_Wheel[x;y;z][m])
  TrackWidthVehicle/1(TrackWidth_Vehicle[m]) -> TARGET_SELECTION_ACC/3
  Dist_Fellows[m]/1 -> TARGET_SELECTION_ACC/4
  v_Rel_Fellows[m|s]/1 -> TARGET_SELECTION_ACC/5
  Angle_Hor_Rel_Fellows[deg]/1 -> TARGET_SELECTION_ACC/6
  Reset[0|1]/1 -> Map_Inputs/1(Reset[0|1]), USER_INTERFACE_ACC/11, TARGET_SELECTION_ACC/7
  d_Total_Fellows[m]/1 -> TARGET_SELECTION_ACC/9
  s_Fellows_Ref[m]/1 -> Rate Transition1/1
  s_Vehicle_Road[m]/1 -> TARGET_SELECTION_ACC/10
  d_Vehicle_Road[m]/1 -> TARGET_SELECTION_ACC/11
  Object_ID[]/1 -> TARGET_SELECTION_ACC/16
  TARGET_SELECTION_ACC/5 -> CONTROLLER_ACC/5
  TARGET_SELECTION_ACC/6 -> CONTROLLER_ACC/6
  Length_Fellows[m]/1 -> TARGET_SELECTION_ACC/13
  Width_Fellows[m]/1 -> TARGET_SELECTION_ACC/14
  Height_Fellows[m]/1 -> TARGET_SELECTION_ACC/15
  PosVec_MainPnt_Fellows[x;y;z][m]/1 -> Input_Selection/1(PosVec_MainPnt_Fellows[x;y;z][m])
  Input_Selection/1(Pos_x_MainPnt_Fellows[m]) -> TARGET_SELECTION_ACC/12
  Rate Transition1/1 -> TARGET_SELECTION_ACC/8
  OUTPUT_INTERFACE_ACC/4 -> Trq_Request_Engine_ACC[Front;Rear][Nm]/1
  TrqDistri_Front_Rear[0_1]/1 -> OUTPUT_INTERFACE_ACC/13
  i_FrontDrive[]/1 -> Mux/1
  i_RearDrive[]/1 -> Mux/2
  ControlModel_Signals/1(ACC_State[1OFF|2Standby|3ON]) -> ACC_State[1OFF|2Standby|3ON]/1
  ControlModel_Signals/2(Driver_Override_ACC_Active[0Off|1On]) -> Driver_Override_ACC_Active[0Off|1On]/1
  ControlModel_Signals/3(Driver_Override_ACC_Reason[0NoOverride|1BrakePedal|2AccPedal]) -> Driver_Override_ACC_Reason[0NoOverride|1BrakePedal|2AccPedal]/1

== system ASM_Traffic_MultiCore/DomainControl/DriverAssistance/Control/Sw_ECU_Signals/ACC_State[1OFF|2Standby|3ON] ==
  SoftECU : Inport
  RealECU : Inport  Port=2
  Const_ACC_State[1OFF|2Standby|3ON] : Constant
  MultiPortSwitch : MultiPortSwitch
  Sw_ACC_State[1SoftECU|2RealECU|3Const] : Constant  Value=CPT.MDL_SW.Sw_ACC_State.v
  ACC_State[1OFF|2Standby|3ON] : Outport  VectorParamsAs1DForOutWhenUnconnected=off
  wires:
  MultiPortSwitch/1 -> ACC_State[1OFF|2Standby|3ON]/1
  Const_ACC_State[1OFF|2Standby|3ON]/1 -> MultiPortSwitch/4
  RealECU/1 -> MultiPortSwitch/3
  SoftECU/1 -> MultiPortSwitch/2
  Sw_ACC_State[1SoftECU|2RealECU|3Const]/1 -> MultiPortSwitch/1

== system ASM_Traffic_MultiCore/DomainControl/DriverAssistance/Control/Sw_ECU_Signals/AEB[0|1] ==
  SoftECU : Inport
  RealECU : Inport  Port=2
  Const_AEB[0|1] : Constant  Value=0
  MultiPortSwitch : MultiPortSwitch
  Sw_AEB[1SoftECU|2RealECU|3Const] : Constant  Value=CPT.MDL_SW.Sw_AEB.v
  AEB[0|1] : Outport  VectorParamsAs1DForOutWhenUnconnected=off
  wires:
  MultiPortSwitch/1 -> AEB[0|1]/1
  Const_AEB[0|1]/1 -> MultiPortSwitch/4
  RealECU/1 -> MultiPortSwitch/3
  SoftECU/1 -> MultiPortSwitch/2
  Sw_AEB[1SoftECU|2RealECU|3Const]/1 -> MultiPortSwitch/1

== system ASM_Traffic_MultiCore/DomainControl/DriverAssistance/Control/Sw_ECU_Signals/Enable_Trq_Decrease_ACC[0|1] ==
  SoftECU : Inport
  RealECU : Inport  Port=2
  Const_Enable_Trq_Decrease_ACC[0|1] : Constant  Value=0
  MultiPortSwitch : MultiPortSwitch
  Sw_Enable_Trq_Decrease_ACC[1SoftECU|2RealECU|3Const] : Constant  Value=CPT.MDL_SW.Sw_Enable_Trq_Decrease_ACC.v
  Enable_Trq_Decrease_ACC[0|1] : Outport  VectorParamsAs1DForOutWhenUnconnected=off
  wires:
  MultiPortSwitch/1 -> Enable_Trq_Decrease_ACC[0|1]/1
  Const_Enable_Trq_Decrease_ACC[0|1]/1 -> MultiPortSwitch/4
  RealECU/1 -> MultiPortSwitch/3
  SoftECU/1 -> MultiPortSwitch/2
  Sw_Enable_Trq_Decrease_ACC[1SoftECU|2RealECU|3Const]/1 -> MultiPortSwitch/1

== system ASM_Traffic_MultiCore/DomainControl/DriverAssistance/Control/Sw_ECU_Signals/Enable_Trq_Increase_ACC[0|1] ==
  SoftECU : Inport
  RealECU : Inport  Port=2
  Const_Enable_Trq_Increase_ACC[0|1] : Constant  Value=0
  MultiPortSwitch : MultiPortSwitch
  Sw_Enable_Trq_Increase_ACC[1SoftECU|2RealECU|3Const] : Constant  Value=CPT.MDL_SW.Sw_Enable_Trq_Increase_ACC.v
  Enable_Trq_Increase_ACC[0|1] : Outport  VectorParamsAs1DForOutWhenUnconnected=off
  wires:
  Sw_Enable_Trq_Increase_ACC[1SoftECU|2RealECU|3Const]/1 -> MultiPortSwitch/1
  SoftECU/1 -> MultiPortSwitch/2
  RealECU/1 -> MultiPortSwitch/3
  Const_Enable_Trq_Increase_ACC[0|1]/1 -> MultiPortSwitch/4
  MultiPortSwitch/1 -> Enable_Trq_Increase_ACC[0|1]/1

== system ASM_Traffic_MultiCore/DomainControl/DriverAssistance/Control/Sw_ECU_Signals/FCW[0|1] ==
  SoftECU : Inport
  RealECU : Inport  Port=2
  Const_FCW[0|1] : Constant  Value=0
  MultiPortSwitch : MultiPortSwitch
  Sw_FCW[1SoftECU|2RealECU|3Const] : Constant  Value=CPT.MDL_SW.Sw_FCW.v
  FCW[0|1] : Outport  VectorParamsAs1DForOutWhenUnconnected=off
  wires:
  MultiPortSwitch/1 -> FCW[0|1]/1
  Const_FCW[0|1]/1 -> MultiPortSwitch/4
  RealECU/1 -> MultiPortSwitch/3
  SoftECU/1 -> MultiPortSwitch/2
  Sw_FCW[1SoftECU|2RealECU|3Const]/1 -> MultiPortSwitch/1

== system ASM_Traffic_MultiCore/DomainControl/DriverAssistance/Control/Sw_ECU_Signals/Trq_DecreaseRequest_ACC[Nm] ==
  SoftECU : Inport
  RealECU : Inport  Port=2
  Const_Trq_DecreaseRequest_ACC[Nm] : Constant  Value=0
  MultiPortSwitch : MultiPortSwitch
  Sw_Trq_DecreaseRequest_ACC[1SoftECU|2RealECU|3Const] : Constant  Value=CPT.MDL_SW.Sw_Trq_DecreaseRequest_ACC.v
  Trq_DecreaseRequest_ACC[Nm] : Outport  VectorParamsAs1DForOutWhenUnconnected=off
  wires:
  MultiPortSwitch/1 -> Trq_DecreaseRequest_ACC[Nm]/1
  Const_Trq_DecreaseRequest_ACC[Nm]/1 -> MultiPortSwitch/4
  RealECU/1 -> MultiPortSwitch/3
  SoftECU/1 -> MultiPortSwitch/2
  Sw_Trq_DecreaseRequest_ACC[1SoftECU|2RealECU|3Const]/1 -> MultiPortSwitch/1

== system ASM_Traffic_MultiCore/DomainControl/DriverAssistance/Control/Sw_ECU_Signals/Trq_IncreaseRequest_ACC[Front;Rear][Nm] ==
  SoftECU : Inport
  RealECU : Inport  Port=2
  Const_Trq_IncreaseRequest_ACC[Front;Rear][Nm] : Constant  Value=[0;0]
  MultiPortSwitch : MultiPortSwitch
  Sw_Trq_IncreaseRequest_ACC[Front;Rear][1SoftECU|2RealECU|3Const] : Constant  Value=CPT.MDL_SW.Sw_Trq_IncreaseRequest_ACC.v
  Trq_IncreaseRequest_ACC[Front;Rear][Nm] : Outport  VectorParamsAs1DForOutWhenUnconnected=off
  wires:
  Sw_Trq_IncreaseRequest_ACC[Front;Rear][1SoftECU|2RealECU|3Const]/1 -> MultiPortSwitch/1
  SoftECU/1 -> MultiPortSwitch/2
  RealECU/1 -> MultiPortSwitch/3
  Const_Trq_IncreaseRequest_ACC[Front;Rear][Nm]/1 -> MultiPortSwitch/4
  MultiPortSwitch/1 -> Trq_IncreaseRequest_ACC[Front;Rear][Nm]/1

== system ASM_Traffic_MultiCore/DomainControl/DriverAssistance/Control/Sw_ECU_Signals/Trq_IncreaseRequest_ACC[Nm] ==
  SoftECU : Inport
  RealECU : Inport  Port=2
  Const_Trq_IncreaseRequest_ACC[Nm] : Constant  Value=0
  MultiPortSwitch : MultiPortSwitch
  Sw_Trq_IncreaseRequest_ACC[1SoftECU|2RealECU|3Const] : Constant  Value=CPT.MDL_SW.Sw_Trq_IncreaseRequest_ACC.v
  Trq_IncreaseRequest_ACC[Nm] : Outport  VectorParamsAs1DForOutWhenUnconnected=off
  wires:
  Sw_Trq_IncreaseRequest_ACC[1SoftECU|2RealECU|3Const]/1 -> MultiPortSwitch/1
  SoftECU/1 -> MultiPortSwitch/2
  RealECU/1 -> MultiPortSwitch/3
  Const_Trq_IncreaseRequest_ACC[Nm]/1 -> MultiPortSwitch/4
  MultiPortSwitch/1 -> Trq_IncreaseRequest_ACC[Nm]/1

== system ASM_Traffic_MultiCore/DomainControl/DriverAssistance/Control/UserInterface/ASMSignalBus_Control ==
  In : Inport
  Terminator_1 : Terminator
  tag scope: ASMBUS_DriverAssistance_Control=global
  wires:
  [ASMBUS_DriverAssistance_Control] -> Terminator_1/1
  In/1 -> [ASMBUS_DriverAssistance_Control]  "Control"

== system ASM_Traffic_MultiCore/DomainControl/DriverAssistance/Control/UserInterface/DISP_Control ==
  Interface_In : Inport
  In : Inport  Port=2
  ACC_Control_Mode[0OFF|1CC|2DC] : Subsystem
      mask Display: disp('')
  ACC_State[0OFF|2Standby|3ON] : Subsystem
      mask Display: disp('')
  AEB[0Off|1On] : Subsystem
      mask Display: disp('')
  Bus Selector1 : BusSelector  OutputSignals=Controller_ACC.State_ACC[0Off|1On],Controller_ACC.Control_Mode_ACC[0Off|1CC|2DC],Controller_ACC.FCW[0Off|1On],Controller_ACC.AEB[0Off|1On],Controller_ACC.TTC[s],Controller_ACC.Collision[0Off|1On],Controller_ACC.Sw_BrakeMode[1Comfort|2AEBOnly|3AEBOff]
  Bus Selector3 : BusSelector  OutputSignals=Controller_ACC.Control_Mode_ACC[0Off|1CC|2DC],Controller_ACC.v_Set[km|h],Target_Selection_ACC.v_Rel[m|s],Controller_ACC.Distance_Set[m],Target_Selection_ACC.Dist_Long[m],Interface_ACC.Trq_Request_Brake_ACC[Nm],Interface_ACC.Trq_Request_Engine_ACC[Nm],Operator_Interface_ACC.ACC_State[1OFF|2Standby|3ON],Target_Selection_ACC.Target_Detected[0|1]
  Bus Selector5 : BusSelector  OutputSignals=ExternalModel.v_Vehicle[km|h]
  Collision[0Off|1On] : Subsystem
      mask Display: disp('')
  Control_Mode_ACC[0Off|1CC|2DC] : Subsystem
      mask Display: disp('')
  Dist_Long[m] : Subsystem
      mask Display: disp('')
  Distance_Set[m] : Subsystem
      mask Display: disp('')
  FCW[0Off|1On] : Subsystem
      mask Display: disp('')
  Mux1 : Mux  Inputs=2
  Mux3 : Mux  Inputs=2
  SoftECU_ACC_Info : Scope  NumInputPorts=6
      settings: TimeSpan=5  ActiveDisplayYMinimum=-0.25  ActiveDisplayYMaximum=2.25  DataLoggingMaxPoints=20000  DataLoggingDecimation=10
  SoftECU_ACC_States : Scope  NumInputPorts=7
      settings: TimeSpan=5  ActiveDisplayYMinimum=-0.125  ActiveDisplayYMaximum=1.125  DataLoggingMaxPoints=20000  DataLoggingDecimation=10  DataLoggingVariableName=ScopeData2
  State_ACC[0Off|1On] : Subsystem
      mask Display: disp('')
  Sw_BrakeMode[1Comfort|2AEBOnly|3AEBOff] : Subsystem
      mask Display: disp('')
  TTC[s] : Subsystem
      mask Display: disp('')
  Target_Detected[0|1] : Subsystem
      mask Display: disp('')
  Terminator : Terminator
  Terminator1 : Terminator
  Trq_Request_Brake_ACC[Nm] : Subsystem
      mask Display: disp('')
  Trq_Request_Engine_ACC[Nm] : Subsystem
      mask Display: disp('')
  UnitConversion : ASM_Utils_lib/UnitConversion/UnitConversion  Selection=m/s_to_km/h
  v_Rel[km|h] : Subsystem
      mask Display: disp('')
  v_Set[km|h] : Subsystem
      mask Display: disp('')
  wires:
  Bus Selector5/1 -> Mux3/2  "<v_Vehicle[km|h]>"
  Bus Selector1/2 -> Control_Mode_ACC[0Off|1CC|2DC]/1(In1)  "<Control_Mode_ACC[0Off|1CC|2DC]>"
  Trq_Request_Engine_ACC[Nm]/1(Out1) -> SoftECU_ACC_Info/6  "Trq_Request_Engine_ACC[Nm]"
  Bus Selector1/5 -> TTC[s]/1(In1)  "<TTC[s]>"
  Bus Selector1/6 -> Collision[0Off|1On]/1(In1)  "<Collision[0Off|1On]>"
  Bus Selector1/4 -> AEB[0Off|1On]/1(In1)  "<AEB[0Off|1On]>"
  Control_Mode_ACC[0Off|1CC|2DC]/1(Out1) -> SoftECU_ACC_States/2  "Control_Mode_ACC[0Off|1CC|2DC]"
  Bus Selector3/2 -> v_Set[km|h]/1(In1)  "<v_Set[km|h]>"
  State_ACC[0Off|1On]/1(Out1) -> SoftECU_ACC_States/1  "State_ACC[0Off|1On]"
  Bus Selector1/3 -> FCW[0Off|1On]/1(In1)  "<FCW[0Off|1On]>"
  FCW[0Off|1On]/1(Out1) -> SoftECU_ACC_States/3  "FCW[0Off|1On]"
  In/1 -> Bus Selector3/1, Bus Selector1/1
  Bus Selector1/7 -> Sw_BrakeMode[1Comfort|2AEBOnly|3AEBOff]/1(In1)  "<Sw_BrakeMode[1Comfort|2AEBOnly|3AEBOff]>"
  AEB[0Off|1On]/1(Out1) -> SoftECU_ACC_States/4  "AEB[0Off|1On]"
  Bus Selector3/3 -> UnitConversion/1  "<v_Rel[m|s]>"
  Trq_Request_Brake_ACC[Nm]/1(Out1) -> SoftECU_ACC_Info/5  "Trq_Request_Brake_ACC[Nm]"
  TTC[s]/1(Out1) -> SoftECU_ACC_States/5  "TTC[s]"
  v_Rel[km|h]/1(Out1) -> SoftECU_ACC_Info/3  "v_Rel[km|h]"
  Mux1/1 -> SoftECU_ACC_Info/4  "Distance[m]"
  Bus Selector3/4 -> Distance_Set[m]/1(In1)  "<Distance_Set[m]>"
  v_Set[km|h]/1(Out1) -> Mux3/1
  Bus Selector3/1 -> ACC_Control_Mode[0OFF|1CC|2DC]/1(In1)  "<Control_Mode_ACC[0Off|1CC|2DC]>"
  Bus Selector3/5 -> Dist_Long[m]/1(In1)  "<Dist_Long[m]>"
  Mux3/1 -> SoftECU_ACC_Info/2  "Velocity[km|h]"
  Sw_BrakeMode[1Comfort|2AEBOnly|3AEBOff]/1(Out1) -> SoftECU_ACC_States/7  "Sw_BrakeMode[1Comfort|2AEBOnly|3AEBOff]"
  UnitConversion/1 -> v_Rel[km|h]/1(In1)
  Bus Selector3/6 -> Trq_Request_Brake_ACC[Nm]/1(In1)  "<Trq_Request_Brake_ACC[Nm]>"
  Distance_Set[m]/1(Out1) -> Mux1/1
  Target_Detected[0|1]/1(Out1) -> Terminator1/1
  Bus Selector3/7 -> Trq_Request_Engine_ACC[Nm]/1(In1)  "<Trq_Request_Engine_ACC[Nm]>"
  Interface_In/1 -> Bus Selector5/1
  Bus Selector1/1 -> State_ACC[0Off|1On]/1(In1)  "<State_ACC[0Off|1On]>"
  Dist_Long[m]/1(Out1) -> Mux1/2
  Collision[0Off|1On]/1(Out1) -> SoftECU_ACC_States/6  "Collision[0Off|1On]"
  ACC_State[0OFF|2Standby|3ON]/1(Out1) -> Terminator/1
  Bus Selector3/9 -> Target_Detected[0|1]/1(In1)  "<Target_Detected[0|1]>"
  Bus Selector3/8 -> ACC_State[0OFF|2Standby|3ON]/1(In1)  "<ACC_State[1OFF|2Standby|3ON]>"
  ACC_Control_Mode[0OFF|1CC|2DC]/1(Out1) -> SoftECU_ACC_Info/1  "ACC_Control_Mode[0OFF|1CC|2DC]"

== system ASM_Traffic_MultiCore/DomainControl/DriverAssistance/Control/UserInterface/PAR_Control ==
  Bus Creator : BusCreator  Inputs=1
  Bus Creator1 : BusCreator  Inputs=9
  Bus Creator2 : BusCreator  Inputs=1
  Sw_ACC_BrakeMode[1Comfort|2AEBOnly|3AEBOff] : Constant  Value=3
  Sw_ACC_Cancel[0Off|1On] : Constant  Value=0
  Sw_ACC_Control_Mode[1ManSched|2Manual] : Constant
  Sw_ACC_Off[0Off|1On] : Constant  Value=0
  Sw_ACC_On[0Off|1On] : Constant  Value=0
  Sw_ACC_Resume[0Off|1On] : Constant  Value=0
  Sw_ACC_Speed_Decrease[0Off|1On] : Constant  Value=0
  Sw_ACC_Speed_Increase[0Off|1On] : Constant  Value=0
  Sw_ACC_Speed_Set[0Off|1On] : Constant  Value=0
  Out : Outport  VectorParamsAs1DForOutWhenUnconnected=off
  wires:
  Sw_ACC_Resume[0Off|1On]/1 -> Bus Creator1/5  "Sw_ACC_Resume[0Off|1On]"
  Sw_ACC_Off[0Off|1On]/1 -> Bus Creator1/3  "Sw_ACC_Off[0Off|1On]"
  Bus Creator1/1 -> Bus Creator/1  "Switches_ACC"
  Sw_ACC_Speed_Increase[0Off|1On]/1 -> Bus Creator1/7  "Sw_ACC_Speed_Increase[0Off|1On]"
  Sw_ACC_On[0Off|1On]/1 -> Bus Creator1/2  "Sw_ACC_On[Off|1On]"
  Bus Creator/1 -> Bus Creator2/1  "SoftECU_ACC"
  Sw_ACC_Cancel[0Off|1On]/1 -> Bus Creator1/4  "Sw_ACC_Cancel[0Off|1On]"
  Sw_ACC_Control_Mode[1ManSched|2Manual]/1 -> Bus Creator1/1  "Sw_ACC_Control_Mode[1ManSched|2Manual]"
  Sw_ACC_Speed_Set[0Off|1On]/1 -> Bus Creator1/6  "Sw_ACC_Speed_Set[0Off|1On]"
  Sw_ACC_Speed_Decrease[0Off|1On]/1 -> Bus Creator1/8  "Sw_ACC_Speed_Decrease[0Off|1On]"
  Sw_ACC_BrakeMode[1Comfort|2AEBOnly|3AEBOff]/1 -> Bus Creator1/9  "Sw_ACC_BrakeMode[1Comfort|2AEBOnly|3AEBOff]"
  Bus Creator2/1 -> Out/1

== system ASM_Traffic_MultiCore/DomainControl/DriverAssistance/Interface_In/ExternalSignals/ExternalECU_ACC ==
  Enable_Trq_Increase_ACC[0|1] : Inport
  Trq_IncreaseRequest_ACC[Nm] : Inport  Port=2
  Trq_IncreaseRequest_ACC[Front;Rear][Nm] : Inport  Port=3
  Enable_Trq_Decrease_ACC[0|1] : Inport  Port=4
  Trq_DecreaseRequest_ACC[Nm] : Inport  Port=5
  FCW[0|1] : Inport  Port=6
  AEB[0|1] : Inport  Port=7
  ACC_State[1OFF|2Standby|3ON] : Inport  Port=8
  Bus Creator : BusCreator  Inputs=8
  Out : Outport  VectorParamsAs1DForOutWhenUnconnected=off
  wires:
  ACC_State[1OFF|2Standby|3ON]/1 -> Bus Creator/8  "ACC_State[1OFF|2Standby|3ON]"
  Trq_IncreaseRequest_ACC[Front;Rear][Nm]/1 -> Bus Creator/3  "Trq_IncreaseRequest_ACC[Front;Rear][Nm]"
  Bus Creator/1 -> Out/1  "ExternalECU"
  Enable_Trq_Increase_ACC[0|1]/1 -> Bus Creator/1  "Enable_Trq_Increase_ACC[0|1]"
  Trq_IncreaseRequest_ACC[Nm]/1 -> Bus Creator/2  "Trq_IncreaseRequest_ACC[Nm]"
  Enable_Trq_Decrease_ACC[0|1]/1 -> Bus Creator/4  "Enable_Trq_Decrease_ACC[0|1]"
  Trq_DecreaseRequest_ACC[Nm]/1 -> Bus Creator/5  "Trq_DecreaseRequest_ACC[Nm]"
  FCW[0|1]/1 -> Bus Creator/6  "FCW[0|1]"
  AEB[0|1]/1 -> Bus Creator/7  "AEB[0|1]"

== system ASM_Traffic_MultiCore/DomainControl/DriverAssistance/Interface_In/ModelSignals/Angle_Hor_Rel_Fellows[deg]_ ==
  In1 : Inport
  Gain : Gain  SaturateOnIntegerOverflow=on  OutDataTypeStr=Inherit: Same as input  ParamDataTypeStr=Inherit: Same as input
  Out1 : Outport  VectorParamsAs1DForOutWhenUnconnected=off
  wires:
  In1/1 -> Gain/1
  Gain/1 -> Out1/1

== system ASM_Traffic_MultiCore/DomainControl/DriverAssistance/Interface_In/ModelSignals/Coef_RollingRes[FL;FR;RL;RR][]_ ==
  In1 : Inport
  Gain : Gain  SaturateOnIntegerOverflow=on  OutDataTypeStr=Inherit: Same as input  ParamDataTypeStr=Inherit: Same as input
  Out1 : Outport  VectorParamsAs1DForOutWhenUnconnected=off
  wires:
  In1/1 -> Gain/1
  Gain/1 -> Out1/1

== system ASM_Traffic_MultiCore/DomainControl/DriverAssistance/Interface_In/ModelSignals/Cw_x[]_ ==
  In1 : Inport
  Gain : Gain  SaturateOnIntegerOverflow=on  OutDataTypeStr=Inherit: Same as input  ParamDataTypeStr=Inherit: Same as input
  Out1 : Outport  VectorParamsAs1DForOutWhenUnconnected=off
  wires:
  In1/1 -> Gain/1
  Gain/1 -> Out1/1

== system ASM_Traffic_MultiCore/DomainControl/DriverAssistance/Interface_In/ModelSignals/Dist_Fellows[m]_ ==
  In1 : Inport
  Gain : Gain  SaturateOnIntegerOverflow=on  OutDataTypeStr=Inherit: Same as input  ParamDataTypeStr=Inherit: Same as input
  Out1 : Outport  VectorParamsAs1DForOutWhenUnconnected=off
  wires:
  In1/1 -> Gain/1
  Gain/1 -> Out1/1

== system ASM_Traffic_MultiCore/DomainControl/DriverAssistance/Interface_In/ModelSignals/ECU_Commands[]_ ==
  In1 : Inport
  Gain : Gain  SaturateOnIntegerOverflow=on  OutDataTypeStr=Inherit: Same as input  ParamDataTypeStr=Inherit: Same as input
  Out1 : Outport  VectorParamsAs1DForOutWhenUnconnected=off
  wires:
  In1/1 -> Gain/1
  Gain/1 -> Out1/1

== system ASM_Traffic_MultiCore/DomainControl/DriverAssistance/Interface_In/ModelSignals/Height_Fellows[m]_ ==
  In1 : Inport
  Gain : Gain  SaturateOnIntegerOverflow=on  OutDataTypeStr=Inherit: Same as input  ParamDataTypeStr=Inherit: Same as input
  Out1 : Outport  VectorParamsAs1DForOutWhenUnconnected=off
  wires:
  In1/1 -> Gain/1
  Gain/1 -> Out1/1

== system ASM_Traffic_MultiCore/DomainControl/DriverAssistance/Interface_In/ModelSignals/Length_Fellows[m]_ ==
  In1 : Inport
  Gain : Gain  SaturateOnIntegerOverflow=on  OutDataTypeStr=Inherit: Same as input  ParamDataTypeStr=Inherit: Same as input
  Out1 : Outport  VectorParamsAs1DForOutWhenUnconnected=off
  wires:
  In1/1 -> Gain/1
  Gain/1 -> Out1/1

== system ASM_Traffic_MultiCore/DomainControl/DriverAssistance/Interface_In/ModelSignals/Object_ID[]_ ==
  In1 : Inport
  Gain : Gain  SaturateOnIntegerOverflow=on  OutDataTypeStr=Inherit: Same as input  ParamDataTypeStr=Inherit: Same as input
  Out1 : Outport  VectorParamsAs1DForOutWhenUnconnected=off
  wires:
  In1/1 -> Gain/1
  Gain/1 -> Out1/1

== system ASM_Traffic_MultiCore/DomainControl/DriverAssistance/Interface_In/ModelSignals/PosVec_MainPnt_Fellows[x;y;z][m]_ ==
  In1 : Inport
  Gain : Gain  SaturateOnIntegerOverflow=on  OutDataTypeStr=Inherit: Same as input  ParamDataTypeStr=Inherit: Same as input
  Out1 : Outport  VectorParamsAs1DForOutWhenUnconnected=off
  wires:
  In1/1 -> Gain/1
  Gain/1 -> Out1/1

== system ASM_Traffic_MultiCore/DomainControl/DriverAssistance/Interface_In/ModelSignals/Pos_AccPedal[%]_ ==
  In1 : Inport
  Gain : Gain  SaturateOnIntegerOverflow=on  OutDataTypeStr=Inherit: Same as input  ParamDataTypeStr=Inherit: Same as input
  Out1 : Outport  VectorParamsAs1DForOutWhenUnconnected=off
  wires:
  In1/1 -> Gain/1
  Gain/1 -> Out1/1

== system ASM_Traffic_MultiCore/DomainControl/DriverAssistance/Interface_In/ModelSignals/Pos_BrakePedal[%]_ ==
  In1 : Inport
  Gain : Gain  SaturateOnIntegerOverflow=on  OutDataTypeStr=Inherit: Same as input  ParamDataTypeStr=Inherit: Same as input
  Out1 : Outport  VectorParamsAs1DForOutWhenUnconnected=off
  wires:
  In1/1 -> Gain/1
  Gain/1 -> Out1/1

== system ASM_Traffic_MultiCore/DomainControl/DriverAssistance/Interface_In/ModelSignals/Pos_FL_Wheel[x;y;z][m]_ ==
  In1 : Inport
  Gain : Gain  SaturateOnIntegerOverflow=on  OutDataTypeStr=Inherit: Same as input  ParamDataTypeStr=Inherit: Same as input
  Out1 : Outport  VectorParamsAs1DForOutWhenUnconnected=off
  wires:
  In1/1 -> Gain/1
  Gain/1 -> Out1/1

== system ASM_Traffic_MultiCore/DomainControl/DriverAssistance/Interface_In/ModelSignals/Pos_FR_Wheel[x;y;z][m]_ ==
  In1 : Inport
  Gain : Gain  SaturateOnIntegerOverflow=on  OutDataTypeStr=Inherit: Same as input  ParamDataTypeStr=Inherit: Same as input
  Out1 : Outport  VectorParamsAs1DForOutWhenUnconnected=off
  wires:
  In1/1 -> Gain/1
  Gain/1 -> Out1/1

== system ASM_Traffic_MultiCore/DomainControl/DriverAssistance/Interface_In/ModelSignals/Reset[0|1]_ ==
  In1 : Inport
  Gain : Gain  SaturateOnIntegerOverflow=on  OutDataTypeStr=Inherit: Same as input  ParamDataTypeStr=Inherit: Same as input
  Out1 : Outport  VectorParamsAs1DForOutWhenUnconnected=off
  wires:
  In1/1 -> Gain/1
  Gain/1 -> Out1/1

== system ASM_Traffic_MultiCore/DomainControl/DriverAssistance/Interface_In/ModelSignals/Slope_Veh_Road[%]_ ==
  In1 : Inport
  Gain : Gain  SaturateOnIntegerOverflow=on  OutDataTypeStr=Inherit: Same as input  ParamDataTypeStr=Inherit: Same as input
  Out1 : Outport  VectorParamsAs1DForOutWhenUnconnected=off
  wires:
  In1/1 -> Gain/1
  Gain/1 -> Out1/1

== system ASM_Traffic_MultiCore/DomainControl/DriverAssistance/Interface_In/ModelSignals/Sw_ModelDeskPlottingInterface[0Disabled|1Enabled]_ ==
  In1 : Inport
  Gain : Gain
  Out1 : Outport
  wires:
  Gain/1 -> Out1/1
  In1/1 -> Gain/1

== system ASM_Traffic_MultiCore/DomainControl/DriverAssistance/Interface_In/ModelSignals/Sw_ModelPortBlocks[0Disabled|1Enabled]_ ==
  In1 : Inport
  Gain : Gain
  Out1 : Outport
  wires:
  Gain/1 -> Out1/1
  In1/1 -> Gain/1

== system ASM_Traffic_MultiCore/DomainControl/DriverAssistance/Interface_In/ModelSignals/TrqDistri_Front_Rear[0_1][]_ ==
  In1 : Inport
  Gain : Gain  SaturateOnIntegerOverflow=on  OutDataTypeStr=Inherit: Same as input  ParamDataTypeStr=Inherit: Same as input
  Out1 : Outport  VectorParamsAs1DForOutWhenUnconnected=off
  wires:
  In1/1 -> Gain/1
  Gain/1 -> Out1/1

== system ASM_Traffic_MultiCore/DomainControl/DriverAssistance/Interface_In/ModelSignals/Trq_Fric_Engine[Nm]_ ==
  In1 : Inport
  Gain : Gain  SaturateOnIntegerOverflow=on  OutDataTypeStr=Inherit: Same as input  ParamDataTypeStr=Inherit: Same as input
  Out1 : Outport  VectorParamsAs1DForOutWhenUnconnected=off
  wires:
  In1/1 -> Gain/1
  Gain/1 -> Out1/1

== system ASM_Traffic_MultiCore/DomainControl/DriverAssistance/Interface_In/ModelSignals/Width_Fellows[m]_ ==
  In1 : Inport
  Gain : Gain  SaturateOnIntegerOverflow=on  OutDataTypeStr=Inherit: Same as input  ParamDataTypeStr=Inherit: Same as input
  Out1 : Outport  VectorParamsAs1DForOutWhenUnconnected=off
  wires:
  In1/1 -> Gain/1
  Gain/1 -> Out1/1

== system ASM_Traffic_MultiCore/DomainControl/DriverAssistance/Interface_In/ModelSignals/YawRate_Vehicle_CoG[deg|s]_ ==
  In1 : Inport
  Gain : Gain  SaturateOnIntegerOverflow=on  OutDataTypeStr=Inherit: Same as input  ParamDataTypeStr=Inherit: Same as input
  Out1 : Outport  VectorParamsAs1DForOutWhenUnconnected=off
  wires:
  In1/1 -> Gain/1
  Gain/1 -> Out1/1

== system ASM_Traffic_MultiCore/DomainControl/DriverAssistance/Interface_In/ModelSignals/d_Total_Fellows[m]_ ==
  In1 : Inport
  Gain : Gain  SaturateOnIntegerOverflow=on  OutDataTypeStr=Inherit: Same as input  ParamDataTypeStr=Inherit: Same as input
  Out1 : Outport  VectorParamsAs1DForOutWhenUnconnected=off
  wires:
  In1/1 -> Gain/1
  Gain/1 -> Out1/1

== system ASM_Traffic_MultiCore/DomainControl/DriverAssistance/Interface_In/ModelSignals/d_Vehicle_Road[m]_ ==
  In1 : Inport
  Gain : Gain  SaturateOnIntegerOverflow=on  OutDataTypeStr=Inherit: Same as input  ParamDataTypeStr=Inherit: Same as input
  Out1 : Outport  VectorParamsAs1DForOutWhenUnconnected=off
  wires:
  In1/1 -> Gain/1
  Gain/1 -> Out1/1

== system ASM_Traffic_MultiCore/DomainControl/DriverAssistance/Interface_In/ModelSignals/i_FrontDrive[]_ ==
  In1 : Inport
  Gain : Gain  SaturateOnIntegerOverflow=on  OutDataTypeStr=Inherit: Same as input  ParamDataTypeStr=Inherit: Same as input
  Out1 : Outport  VectorParamsAs1DForOutWhenUnconnected=off
  wires:
  In1/1 -> Gain/1
  Gain/1 -> Out1/1
